simulink model "FMS"  (R2018b)
settings: configuration reference "fms_config" (kept outside this file)
values from neighbouring files (symbols this model uses):
  FMS_EXPORT = Simulink.Parameter(FMS_EXPORT_VALUE)    [fms_model_init.m]
  FMS_PARAM = Simulink.Parameter(FMS_PARAM_VALUE)    [fms_model_init.m]
undefined symbols (not defined in the file or in its folder): actuator_cmd, ax_cmd, ay_cmd, az_cmd, cmd_mask, ControlMode, ctrl_mode, DiscIntNeverNeededParam, ext_state, FMS_Cmd, FMS_CONST, home, mode, p_cmd, phi_cmd, PilotMode, psi_rate_cmd, q_cmd, r_cmd, reset, state, status, theta_cmd, throttle_cmd, timestamp, u_cmd, v_cmd, VehicleState, VehicleStatus, VTOLState, w_cmd, wp_consume, wp_current
libraries: simulink x141, FMT_Model_Lib x120, hdlsllib x13
(part 12 of 12)

== matlab function FMS/FMS Commander/Commander/Arm/FW_Mode/Auto/Mission/Mission_SubSystem/Position Command/L1 Control/L1 Reference WP/SearchL1RefWP ==
  data: P1 input; P output; P2 input; P3 input; L1 input; u output
% Find reference waypoint (L1RefWP) on the line segment P1P2 which has 
% L1 distance from vehicle position (P3).
%
% The idea is to calculate the intersection point of a circle with L1 radius
% with the line segment P1P2.
%
% Define P = P1 + u * (P2 - P1), where P is the intersection point.
% Goal is calculating the u, where the valid u is between [0, 1].
%
% Input:
%   P1: start point of segment line
%   P2: start point of segment line
%   P3: circle center point, also is known as the vehicle position
%   L1: the L1 distance
% Output:
%   P: L1 reference waypoint
%   u: scale factor (valid between 0 and 1), -1 means no intersection.
function [P, u] = SearchL1RefWP(P1, P2, P3, L1)

% P1 = (x1, y1), P2 = (x2, y2), P3 = (x3, y3)
x1 = P1(1);
y1 = P1(2);
x2 = P2(1);
y2 = P2(2);
x3 = P3(1);
y3 = P3(2);

% The P is on circle and line segment, which yields:
A = (x2 - x1)^2 + (y2 - y1)^2;
B = 2 * ((x2 - x1)*(x1 - x3) + (y2 - y1)*(y1 - y3));
C = x3^2 + y3^2 + x1^2 + y1^2 - 2*(x3*x1 + y3*y1) - L1^2;
% Check root existence confition if B^2 - 4*A*C >= 0
D = B^2 - 4*A*C;
u = single(-1);
P = single([0 0]);

if D > 0
    % D>0 means we have 2 difference roots, % root is valid only if u is in range of [0, 1]
    u1 = (-B + sqrt(D)) / (2*A);
    u2 = (-B - sqrt(D)) / (2*A);
    
    if (u1>=0 && u1<=1) && (u2>=0 && u2<=1)
        % have 2 valid roots, select the one which is closer to P2 (target point)
        if u1 > u2
            u = u1; 
        else
            u = u2;
        end
    elseif (u1>=0 && u1<=1)
        % only 1 root valid, select it
        u = u1;
    elseif (u2>=0 && u2<=1)
        % only 1 root valid, select it
        u = u2;
    else
        % no valid root, which means no intersection point founded.
        return;
    end
elseif D == 0
    % D=0 means only 1 single root
    u1 = -B / (2*A);
    if (u1>=0 && u1<=1)
        % valid root, select it
        u = u1;
    else
        % no valid root, which means no intersection point founded.
        return;
    end
else
    % no valid root, which means no intersection point founded.
    return;
end

% calculate the L1 reference waypoint (P) coordinate
P(1) = x1 + u*(x2 - x1);
P(2) = y1 + u*(y2 - y1);

== matlab function FMS/FMS Commander/Commander/Arm/FW_Mode/SubMode/Hold/Loiter_Control/L1 Reference WP/OutRegionRegWP ==
  data: P0 input; P output; P_Vehicle input; R input; L1 input; n input
% Find the reference waypoint when vehicle has no intersection with loicter circle.
%
% There are two region defined:
%   Region 1: The vehicle is outside of loiter circle
%   Region 2: The else situation
%
function P = OutRegionRefWP(P0, P_Vehicle, R, L1, n)

if sum((P_Vehicle-P0).^2) > R^2
    % outside of loiter circle, we just select P0 as P
    P = P0;
else
    % inside of loiter circle, we just let vehicle keep current direction
    P = P_Vehicle + n*L1;
end

== matlab function FMS/FMS Commander/Commander/Arm/FW_Mode/SubMode/Hold/Loiter_Control/L1 Reference WP/SearchL1RefWP ==
  data: P_0 input; P output; P_Vehicle input; R input; L1 input; n output
% Find reference waypoint (L1RefWP) on the loiter circle with origin at 
% P_0 and radius of R
%
% The idea is to calculate the intersection point of 2 circles (P_0:R and
% P_Vehicle:L1).
% Refer to: Knut Andreas Lie's Unstructured PEBI-grids Adapting to Geological Features in Subsurface Reservoirs
%
% Input:
%   P_0: loiter circle origin
%   P_Vehicle: vehicle position
%   R: loiter radius
%   L1: the L1 distance
% Output:
%   P: L1 reference waypoint
%   n: number of intersection points.
function [P, n] = SearchL1RefWP(P_0, P_Vehicle, R, L1)

C0 = P_Vehicle;
R0 = L1;
C1 = P_0;
R1 = R;
P = single([0;0]);

if C0(1)==C1(1) && C0(2)==C1(2) && R==L1
   % we have 2 same circle
   n = 0;
   return;
end

d = sqrt(sum((C1-C0).^2));
a = (d^2 + R0^2 - R1^2) / (2*d);

% n1 is perpendicular to n0
n0 = (C1-C0)/d;
n1 = [0 -1; 1 0] * n0;

if a^2 > R0^2
    % no intersection
    n = 0;
elseif a^2 == R0^2
    % only 1 intersection
    n = 1;
    P = C0 + a*n0;
else
    % 2 intersection
    n = 2;
    % we always choose the point with clockwise direction,
    % if wants anti-clockwise direction, choose h = -sqrt(R0^2 - a^2)
    h = sqrt(R0^2 - a^2);
    P = C0 + a*n0 + h*n1; 
end

== matlab function FMS/FMS Commander/Commander/Arm/FW_Mode/SubMode/Return/Position Command/L1 Control/L1 Reference WP/NearbyRefWP ==
  data: P output; P2 input; d output; P3 input; L1 input
% Find the reference waypoint when vehicle (P3) is close to target (P2)
%
% If the vehicle is close to target (distance(P2,P3) < L1), select P2 as
% reference waypoint and return the distance, otherwise return -1.
function [P,d] = NearbyRefWP(P2, P3, L1)

P3P2 = P2 - P3;
dis = sqrt(sum(P3P2.^2));

if dis <= L1
    d = dis;
    % select P2 as reference WP
    P = P2;
else
    d = single(-1);
    % unset WP
    P = single([0; 0]);
end

== matlab function FMS/FMS Commander/Commander/Arm/FW_Mode/SubMode/Return/Position Command/L1 Control/L1 Reference WP/OutRegionRegWP ==
  data: P1 input; P output; P2 input; P3 input; L1 input
% Find the reference waypoint when vehicle is out of L1 region near P1P2.
%
% There are three region defined:
%   Region 1: The project point of P3 is lied on left side of P1P2
%   Region 2: The project point of P3 is lied on right side of P1P2
%   Region 3: The project point of P3 is lied on the segment line 
%
%   For the case of region 3, we select the project point as the reference
%   wayspoint. For the case of region 1, we choose P1 as reference waypoint
%   and similarly for the case of region 2, we choose P2 as reference
%   waypoint.
function P = OutRegionRefWP(P1, P2, P3, L1)
% segment line P1P2
P1P2 = P2 - P1;
% segment line P1P3
P1P3 = P3 - P1;

% Define C as the P3 project point on line P1P2.
% Hence, P1C = dot(P1P3, P1P2)/|P1P2| * (P1P2/|P1P2|) = u * P1P2
% where u = dot(P1P3, P1P2) / |P1P2|^2.
u = dot(P1P3, P1P2) / sum(P1P2.^2);

% if u <= 0
%     % region 1
%     P = P1;
% elseif u >= 1
%     % region 2
%     P = P2;
% else
%     % region 3. C = P1C + P1
%     % P = u * P1P2 + P1;
%     
%     C = u * P1P2 + P1;
%     % tan(pi/6) = 0.5774
%     u = sqrt(sum((C-P3).^2))*single(0.5774)/sqrt(sum(P1P2.^2)) + u;
%     if u > 1
%         u = single(1);
%     end
%     P = u * P1P2 + P1;
% end

if u >= 1
    % region 1: Project is on right side of P2
    P = P2;
else
    % region 2. Project is on left side of P2
    u = L1/sqrt(sum(P1P2.^2)) + u;
    
    if u > 1
        u = single(1);
    elseif u < 0
        u = single(0);
    end
    
    P = u * P1P2 + P1;
end

== matlab function FMS/FMS Commander/Commander/Arm/FW_Mode/SubMode/Return/Position Command/L1 Control/L1 Reference WP/SearchL1RefWP ==
  data: P1 input; P output; P2 input; P3 input; L1 input; u output
% Find reference waypoint (L1RefWP) on the line segment P1P2 which has 
% L1 distance from vehicle position (P3).
%
% The idea is to calculate the intersection point of a circle with L1 radius
% with the line segment P1P2.
%
% Define P = P1 + u * (P2 - P1), where P is the intersection point.
% Goal is calculating the u, where the valid u is between [0, 1].
%
% Input:
%   P1: start point of segment line
%   P2: start point of segment line
%   P3: circle center point, also is known as the vehicle position
%   L1: the L1 distance
% Output:
%   P: L1 reference waypoint
%   u: scale factor (valid between 0 and 1), -1 means no intersection.
function [P, u] = SearchL1RefWP(P1, P2, P3, L1)

% P1 = (x1, y1), P2 = (x2, y2), P3 = (x3, y3)
x1 = P1(1);
y1 = P1(2);
x2 = P2(1);
y2 = P2(2);
x3 = P3(1);
y3 = P3(2);

% The P is on circle and line segment, which yields:
A = (x2 - x1)^2 + (y2 - y1)^2;
B = 2 * ((x2 - x1)*(x1 - x3) + (y2 - y1)*(y1 - y3));
C = x3^2 + y3^2 + x1^2 + y1^2 - 2*(x3*x1 + y3*y1) - L1^2;
% Check root existence confition if B^2 - 4*A*C >= 0
D = B^2 - 4*A*C;
u = single(-1);
P = single([0 0]);

if D > 0
    % D>0 means we have 2 difference roots, % root is valid only if u is in range of [0, 1]
    u1 = (-B + sqrt(D)) / (2*A);
    u2 = (-B - sqrt(D)) / (2*A);
    
    if (u1>=0 && u1<=1) && (u2>=0 && u2<=1)
        % have 2 valid roots, select the one which is closer to P2 (target point)
        if u1 > u2
            u = u1; 
        else
            u = u2;
        end
    elseif (u1>=0 && u1<=1)
        % only 1 root valid, select it
        u = u1;
    elseif (u2>=0 && u2<=1)
        % only 1 root valid, select it
        u = u2;
    else
        % no valid root, which means no intersection point founded.
        return;
    end
elseif D == 0
    % D=0 means only 1 single root
    u1 = -B / (2*A);
    if (u1>=0 && u1<=1)
        % valid root, select it
        u = u1;
    else
        % no valid root, which means no intersection point founded.
        return;
    end
else
    % no valid root, which means no intersection point founded.
    return;
end

% calculate the L1 reference waypoint (P) coordinate
P(1) = x1 + u*(x2 - x1);
P(2) = y1 + u*(y2 - y1);

== matlab function FMS/FMS Commander/Commander/Arm/FW_Mode/SubMode/Takeoff/Position Command/L1 Control/L1 Reference WP/NearbyRefWP ==
  data: P output; P2 input; d output; P3 input; L1 input
% Find the reference waypoint when vehicle (P3) is close to target (P2)
%
% If the vehicle is close to target (distance(P2,P3) < L1), select P2 as
% reference waypoint and return the distance, otherwise return -1.
function [P,d] = NearbyRefWP(P2, P3, L1)

P3P2 = P2 - P3;
dis = sqrt(sum(P3P2.^2));

if dis <= L1
    d = dis;
    % select P2 as reference WP
    P = P2;
else
    d = single(-1);
    % unset WP
    P = single([0; 0]);
end

== matlab function FMS/FMS Commander/Commander/Arm/FW_Mode/SubMode/Takeoff/Position Command/L1 Control/L1 Reference WP/OutRegionRegWP ==
  data: P1 input; P output; P2 input; P3 input
% Find the reference waypoint when vehicle is out of L1 region near P1P2.
%
% There are three region defined:
%   Region 1: The project point of P3 is lied on left side of P1P2
%   Region 2: The project point of P3 is lied on right side of P1P2
%   Region 3: The project point of P3 is lied on the segment line 
%
%   For the case of region 3, we select the project point as the reference
%   wayspoint. For the case of region 1, we choose P1 as reference waypoint
%   and similarly for the case of region 2, we choose P3 as reference
%   waypoint.
function P = OutRegionRefWP(P1, P2, P3)
% segment line P1P2
P1P2 = P2 - P1;
% segment line P1P3
P1P3 = P3 - P1;

% Define C as the P3 project point on line P1P2.
% Hence, P1C = dot(P1P3, P1P2)/|P1P2| * (P1P2/|P1P2|) = u * P1P2
% where u = dot(P1P3, P1P2) / |P1P2|^2.
u = dot(P1P3, P1P2) / sum(P1P2.^2);

if u <= 0
    % region 1
    P = P1;
elseif u >= 1
    % region 2
    P = P2;
else
    % region 3. C = P1C + P1
    % P = u * P1P2 + P1;
    
    C = u * P1P2 + P1;
    % tan(pi/6) = 0.5774
    u = sqrt(sum((C-P3).^2))*single(0.5774)/sqrt(sum(P1P2.^2)) + u;
    if u > 1
        u = single(1);
    end
    P = u * P1P2 + P1;
end

== matlab function FMS/FMS Commander/Commander/Arm/FW_Mode/SubMode/Takeoff/Position Command/L1 Control/L1 Reference WP/SearchL1RefWP ==
  data: P1 input; P output; P2 input; P3 input; L1 input; u output
% Find reference waypoint (L1RefWP) on the line segment P1P2 which has 
% L1 distance from vehicle position (P3).
%
% The idea is to calculate the intersection point of a circle with L1 radius
% with the line segment P1P2.
%
% Define P = P1 + u * (P2 - P1), where P is the intersection point.
% Goal is calculating the u, where the valid u is between [0, 1].
%
% Input:
%   P1: start point of segment line
%   P2: start point of segment line
%   P3: circle center point, also is known as the vehicle position
%   L1: the L1 distance
% Output:
%   P: L1 reference waypoint
%   u: scale factor (valid between 0 and 1), -1 means no intersection.
function [P, u] = SearchL1RefWP(P1, P2, P3, L1)

% P1 = (x1, y1), P2 = (x2, y2), P3 = (x3, y3)
x1 = P1(1);
y1 = P1(2);
x2 = P2(1);
y2 = P2(2);
x3 = P3(1);
y3 = P3(2);

% The P is on circle and line segment, which yields:
A = (x2 - x1)^2 + (y2 - y1)^2;
B = 2 * ((x2 - x1)*(x1 - x3) + (y2 - y1)*(y1 - y3));
C = x3^2 + y3^2 + x1^2 + y1^2 - 2*(x3*x1 + y3*y1) - L1^2;
% Check root existence confition if B^2 - 4*A*C >= 0
D = B^2 - 4*A*C;
u = single(-1);
P = single([0 0]);

if D > 0
    % D>0 means we have 2 difference roots, % root is valid only if u is in range of [0, 1]
    u1 = (-B + sqrt(D)) / (2*A);
    u2 = (-B - sqrt(D)) / (2*A);
    
    if (u1>=0 && u1<=1) && (u2>=0 && u2<=1)
        % have 2 valid roots, select the one which is closer to P2 (target point)
        if u1 > u2
            u = u1; 
        else
            u = u2;
        end
    elseif (u1>=0 && u1<=1)
        % only 1 root valid, select it
        u = u1;
    elseif (u2>=0 && u2<=1)
        % only 1 root valid, select it
        u = u2;
    else
        % no valid root, which means no intersection point founded.
        return;
    end
elseif D == 0
    % D=0 means only 1 single root
    u1 = -B / (2*A);
    if (u1>=0 && u1<=1)
        % valid root, select it
        u = u1;
    else
        % no valid root, which means no intersection point founded.
        return;
    end
else
    % no valid root, which means no intersection point founded.
    return;
end

% calculate the L1 reference waypoint (P) coordinate
P(1) = x1 + u*(x2 - x1);
P(2) = y1 + u*(y2 - y1);

== matlab function FMS/FMS Commander/Commander/Arm/BackwardTrans_Mode/Position Command/Controller/Hold Control/L1_Reference_WP/OutRegionRefWP ==
  data: c input; P output; p0 input; n input
function P  = OutRegionRefWP(c, p0, n)

P1P3 = c - p0;

% Define C as the P3 (vehicle) project point on ray.
% Hence, P1C = dot(P1P3, P1P2)/|P1P2| * (P1P2/|P1P2|) = t * P1P2
% where t = dot(P1P3, P1P2) / |P1P2|^2. Choose P1P2 as a normalized vector,
% therefore |P1P2| = 1, yield t = dot(P1P3, n)
t = dot(P1P3, n);
C = p0 + t*n;

% Now we calculate the distance forward from C with 30deg
d1 = norm(C - c);
d2 = d1 * tan(pi/6);

% Calculate the final waypoint
P = p0 + (t+d2)*n;

== matlab function FMS/FMS Commander/Commander/Arm/BackwardTrans_Mode/Position Command/Controller/Hold Control/L1_Reference_WP/SearchL1RefWP ==
  data: c input; P output; p0 input; n input; L1 input; t output
function [P, t] = SearchL1RefWP(c, p0, n, L1)

m = p0 - c;
A = 1;  % dot(n,n) = 1
B = 2*dot(n, m);
C = dot(m, m) - L1^2;

% Check root existence confition if B^2 - 4*A*C >= 0
D = B^2 - 4*A*C;

t = single(-1);
P = single([0;0]);

if D > 0
    % D>0 means we have 2 difference roots, % root is valid only if u is in range of [0, 1]
    u1 = (-B + sqrt(D)) / (2*A);
    u2 = (-B - sqrt(D)) / (2*A);
    
    % have 2 valid roots, select the one which is farthur
    if u1 > u2
        t = u1; 
    else
        t = u2;
    end
    
    % calculate the L1 reference waypoint (P) coordinate
    P = p0 + t*n;
elseif D == 0
    t = -B / (2*A);
    
    % calculate the L1 reference waypoint (P) coordinate
    P = p0 + t*n;
else
    % only 1 root or no valid root, use other logic to find WP.
    return;
end

== stateflow chart FMS/FMS Commander/Commander/Arm/BackwardTrans_Mode/Position Command/Detect Movement/Motion State ==
  state Hold
    entry:
    state=MotionState.Hold;
  state Move
    entry:
    state=MotionState.Move;
  state Brake
    entry:
    state=MotionState.Brake;
  (default) -> Move
  Hold -> Move : [motion_req==1]
  Brake -> Move [order 2] : [motion_req==1]
  Move -> Brake : [motion_req==0]
  Brake -> Hold [order 1] : [after(2.5, sec) && speed > 5]
  data: state output Enum: MotionState; motion_req input; speed input
